simulink model "SpeedGoatLoop_v2"  (R2020b)
settings: Solver=FixedStepAuto  StartTime=0.0  StopTime=60*60*3  RelTol=1e-3
libraries: fl_lib x45, nesl_utility x19, SimscapeFluids_lib x4, speedgoatlib_IO132 x2, slpidlib x1
settings Model: SimulationMode=external  EnablePacing=on  PacingRate=45  ExtModeEnableFloating=off  Creator=cheap  LastModifiedBy=cheap
settings SolverCC: ConcurrentTasks=on  PositivePriorityOrder=on
settings OptimizationCC: BlockReduction=off  OptimizeBlockIOStorage=off
settings DebuggingCC: TasksWithSamePriorityMsg=none
settings HardwareCC: ProdBitPerLong=64  ProdLongLongMode=on  ProdHWDeviceType=Intel->x86-64 (Linux 64)
settings RTWCC: Description=Simulink Real-Time  SystemTargetFile=slrealtime.tlc  TemplateMakefile=slrealtime_default_tmf  Toolchain=Simulink Real-Time Toolchain  BuildConfiguration=Faster Runs  CodeExecutionProfiling=on  TargetLang=C++

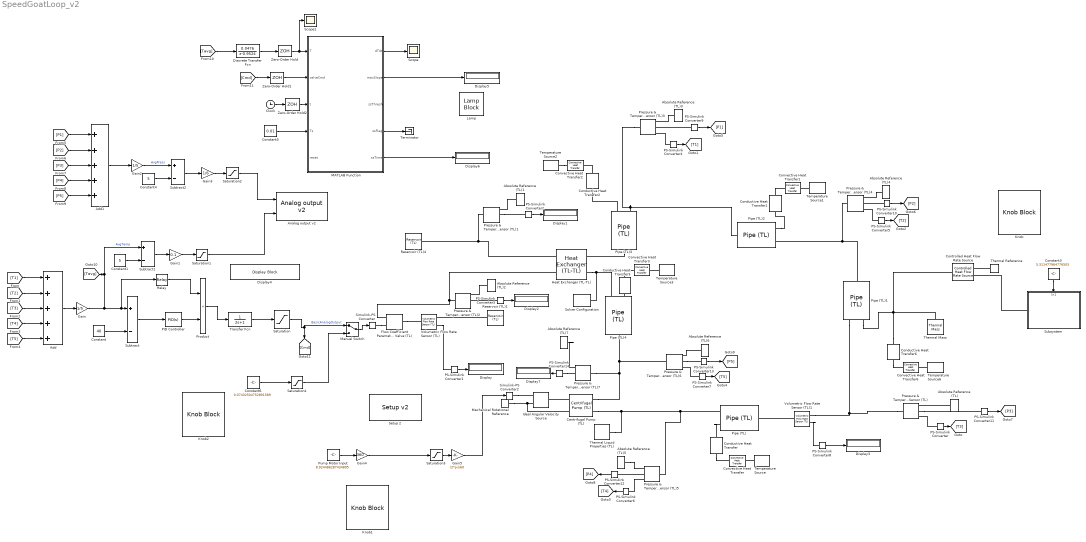
== system SpeedGoatLoop_v2 ==
  Absolute Reference (TL){,1..7} (8 alike) : fl_lib/Thermal Liquid/Elements/Absolute Reference (TL)
      settings: SourceProductBaseCode=SS
  Add : Sum  Inputs=+++++
  Add1 : Sum  Inputs=+++++
  "Analog output v2 " : speedgoatlib_IO132/Analog output v2   parModuleId=1  parSampleTime=-1  parPciSlot=-1  parDacChannels=[1 2]  parDacVoltageRange=[2 2 1 1]  parDacInitValues=[1 1]  parDacReset=[1 1]  parDacSyncOut=1  parDacDmaEnable=0  parDacActiveDmaDevices=1  parDacDmaLatency=2  parDacFrameSize=100
      settings: SourceProductName=Simulink Real-Time: Speedgoat I/O Blockset
  Centrifugal Pump (TL) : SimscapeFluids_lib/Thermal Liquid/Pumps & Motors/Centrifugal Pump (TL)  pump_parameterization=1  mech_orientation=1  flow_rate_1D_TLU=[0 8.33e-5 1.67e-4 2.50e-4 3.33e-4 4.17e-4 5.00e-4 5.83e-4 6.67e-4] m^3/s  head_1D_TLU=[20 19.7 19.0 18.0 16.8 15.2 13.0 10.2 7.5] m  power_1D_TLU=[0 40 80 140 210 290 380 470 550] W  rho_ref_1D=998 kg/m^3  omega_ref_1D=363 rad/s  flow_rate_2D_TLU=[16.67, 23.33, 30, 40, 53.33, 60] lpm  omega_2D_TLU=[2450, 2800, 3150, 3500] rpm  head_2D_TLU=[25, 32.7, 42.5, 50; 24, 31.7, 41, 49; 22.7, 30.5, 39, 47.5; 20, 28, 36, 45; 15.7, 24, 32, 40; 12.5, 21, 29.5, 37.5] m  power_2D_TLU=[.28, .38, .5, .6; .31, .41, .55, .68; .33, .44, .6, .75; .36, .48, .65, .83; .38, .53, .72, .93; .39, .55, .75, .97] kW  rho_ref_2D=920 kg/m^3  omega_threshold=10 rad/s  area=((pi*2)^2)/4 in^2  mdot_A_specify=off  mdot_A_priority=None  mdot_A=1 kg/s  mdot_A_nominal_specify=off  mdot_A_nominal_unit=kg/s  mdot_A_nominal_value=1
      settings: SourceProductBaseCode=SH  InternalSimscapePortConfiguration="{\"Bottom\":[],\"Left\":[{\"id\":\"A\",\"label\":\"A\",\"type\":\"foundation.thermal_liquid.thermal_liquid\"},{\"id\":\"B\",\"label\":\"B\",\"type\":\"foundation.thermal_liquid.thermal_liquid\"}],\"Right\":[{\"id\":\"R\",\"label\":\"R\",\"type\":\"foundation.mechanical.rotational.rotational\"},{\"id\":\"C\",\"label\":\"C\",\"type\":\"foundation.mechanical.rotational.rotational\"}],\"Top\":[]}"
  Clock : Clock
  Conductive Heat Transfer{,1..3,6} (5 alike) : fl_lib/Thermal/Thermal Elements/Conductive Heat Transfer  area=1e-4 m^2  thickness=0.1 m  th_cond=16.2 W/(K*m)  T_specify=off  T_priority=None  T=0 K  T_nominal_specify=off  T_nominal_unit=K  T_nominal_value=1  Q_specify=off  Q_priority=None  Q=0 W  Q_nominal_specify=off  Q_nominal_unit=W  Q_nominal_value=1
  Constant : Constant  Value=40
  Constant1 : Constant  Value=5
  Constant3 : Constant  Value=5.311477964776503
  Constant4 : Constant  Value=5
  Constant5 : Constant  Value=0.01
  Constant6 : Constant  Value=0.07432504752891589
  Controlled Heat Flow Rate Source : fl_lib/Thermal/Thermal Sources/Controlled Heat Flow Rate Source
  Convective Heat Transfer{,1..3} (4 alike) : fl_lib/Thermal/Thermal Elements/Convective Heat Transfer  area=pi*50*(656.10+50.8+179.35+254) mm^2  heat_tr_coeff=10 W/(K*m^2)  T_specify=off  T_priority=None  T=0 K  T_nominal_specify=off  T_nominal_unit=K  T_nominal_value=1  Q_specify=off  Q_priority=None  Q=0 W  Q_nominal_specify=off  Q_nominal_unit=W  Q_nominal_value=1
  Convective Heat Transfer6 : fl_lib/Thermal/Thermal Elements/Convective Heat Transfer  area=pi*50*(6000) mm^2  heat_tr_coeff=10 W/(K*m^2)  T_specify=off  T_priority=None  T=0 K  T_nominal_specify=off  T_nominal_unit=K  T_nominal_value=1  Q_specify=off  Q_priority=None  Q=0 W  Q_nominal_specify=off  Q_nominal_unit=W  Q_nominal_value=1
  Discrete Transfer Fcn : DiscreteTransferFcn  Numerator=[0.0476]  Denominator=[1 -0.9524]  SampleTime=0.01
  Display{,1..3,5..7} (7 alike) : Display
  Display4 : DisplayBlock  LabelPosition=Hide  Format=short  Transparency=1
  Flow Coefficient Parameterized Valve (TL) : SimscapeFluids_lib/Thermal Liquid/Valves & Orifices/Flow Coefficient Parameterized Valve (TL)  flow_coeff_spec=fluids.thermal_liquid.valves.enum.flow_coeff_spec.cv  Cv_max=1  Cv_min=1e-4  Kv_max=1  Kv_min=1e-4  valve_character=fluids.thermal_liquid.valves.enum.valve_opening_spec.linear  rangeability=50  alpha=2  area=((0.75*pi)^2)/4 in^2  length=3 in  Re_c=12  smoothing_factor=0.02  opening_dynamic=simscape.enum.onoff.off  tau=0.1 s  mdot_A_specify=off  mdot_A_priority=None  mdot_A=1 kg/s  mdot_A_nominal_specify=off  mdot_A_nominal_unit=kg/s  mdot_A_nominal_value=1  area_dynamic_specify=off  area_dynamic_priority=High  area_dynamic=1e-10 m^2  area_dynamic_nominal_specify=off  area_dynamic_nominal_unit=m^2  area_dynamic_nominal_value=1
      settings: SourceProductBaseCode=SH  InternalSimscapePortConfiguration="{\"Bottom\":[],\"Left\":[{\"id\":\"A\",\"label\":\"A\",\"type\":\"foundation.thermal_liquid.thermal_liquid\"},{\"id\":\"L\",\"label\":\"L\",\"type\":\"input\"}],\"Right\":[{\"id\":\"B\",\"label\":\"B\",\"type\":\"foundation.thermal_liquid.thermal_liquid\"}],\"Top\":[]}"
  Gain : Gain  Gain=1/5
  Gain1 : Gain  Gain=0.1
  Gain2 : Gain  Gain=1/5
  Gain3 : Gain  Gain=1/6
  Gain4 : Gain  Gain=360
  Gain5 : Gain  Gain=(2*pi)/60
  Heat Exchanger (TL-TL) : SimscapeFluids_lib/Fluid Network Interfaces/Heat Exchangers/Heat Exchanger (TL-TL)  hex_type=fluids.interfaces.enum.flow_arrangement_spec.shell_tube  cross_type=fluids.interfaces.enum.cross_flow_heat_exchanger_TL_TL_spec.mixed_mixed  shell_num=1  NTU_TLU=[.5, 1, 2, 3, 4, 5]  CR_TLU=[0, .25, .5, .75, 1]  eff_TLU=[.3, .3, .3, .3, .3; .6, .55, .5, .47, .43; .85, .76, .68, .61, .55; .94, .83, .72, .65, .58; .98, .86, .75, .66, .58; .99, .86, .75, .66, .58]  wall_thermal_dynamics=simscape.enum.onoff.on  thermal_mass_wall=447 J/K  R_wall=1.984E-3 K/W  min_flow_area_1=1.16E-3 m^2  Dh_press_1=0.00451 m  liquid_volume_1=3E-3 m^3  Re_lam_1=2000  Re_tur_1=4000  pressure_loss_spec_1=fluids.interfaces.enum.pressure_loss_spec.constant  min_flow_area_2=9.19E-4 m^2  Dh_press_2=0.004572 m  liquid_volume_2=8.41E-4 m^3  Re_lam_2=2000  Re_tur_2=4000  pressure_loss_spec_2=fluids.interfaces.enum.pressure_loss_spec.tube_correlation  pressure_loss_coeff_1=0.1  length_press_1=1 m  length_add_1=0.1 m  roughness_1=15e-6 m  Re_friction_TLU_1=[400, 1000, 1500, 3000, 4000, 6000, 10000, 20000, 40000, 60000, 100000, 100000000]  friction_factor_TLU_1=[.264, .112, .071, .0417, .0387, .0268, .025, .0232, .0226, .022, .0214, .0214]  shape_factor_1=64  Re_Euler_TLU_1=[50, 500, 1000, 2000]  Euler_TLU_1=[4.4505, .6864, .4791, .3755]  pressure_loss_coeff_2=0.1  length_press_2=0.9144 m  length_add_2=0.4 m  roughness_2=15e-6 m  Re_friction_TLU_2=[400, 1000, 1500, 3000, 4000, 6000, 10000, 20000, 40000, 60000, 100000, 100000000]  friction_factor_TLU_2=[.264, .112, .071, .0417, .0387, .0268, .025, .0232, .0226, .022, .0214, .0214]  shape_factor_2=64  Re_Euler_TLU_2=[50, 500, 1000, 2000]  Euler_TLU_2=[4.4505, .6864, .4791, .3755]  heat_transfer_spec_1=fluids.interfaces.enum.heat_transfer_spec.constant  heat_transfer_spec_2=fluids.interfaces.enum.heat_transfer_spec.tube_correlation  heat_coeff_1=100 W/(m^2 * K)  length_heat_1=1 m  Nu_lam_1=3.66  Re_Colburn_TLU_1=[100, 150, 1000]  Colburn_factor_TLU_1=[.019, .013, .002]  Re_Nu_TLU_1=[100, 150, 1000]  Pr_Nu_TLU_1=[1, 10]  Nu_TLU_1=[3.72, 4.21; 3.75, 4.44; 4.21, 7.15]  heat_coeff_2=100 W/(m^2 * K)  length_heat_2=0.9144 m  Nu_lam_2=3.66  Re_Colburn_TLU_2=[100, 150, 1000]  Colburn_factor_TLU_2=[.019, .013, .002]  Re_Nu_TLU_2=[100, 150, 1000]  Pr_Nu_TLU_2=[1, 10]  Nu_TLU_2=[3.72, 4.21; 3.75, 4.44; 4.21, 7.15]  heat_transfer_area_1=1.022 m^2  fouling_factor_1=1e-4 m^2*K/W  min_heat_coeff_1=3000 W/(m^2 * K)  heat_transfer_area_2=0.735 m^2  fouling_factor_2=1e-4 m^2*K/W  min_heat_coeff_2=10000 W/(m^2 * K)  dynamic_compressibility_1=simscape.enum.onoff.on  T0_1=10 degC  p0_1=60 psi  dynamic_compressibility_2=simscape.enum.onoff.on  T0_2=24 degC  p0_2=30 psi  mdot1_TLU=[.3, .5, .6, .7, 1, 1.4, 1.9, 2.3] kg/s  mdot2_TLU=[.3, .5, 1, 1.3, 1.7, 2, 2.6, 3.3] kg/s  SD_TLU=[.324, .3533, .404, .4253, .4333, .4373, .4453, .4533; .3813, .424, .496, .5307, .544, .5547, .5693, .5787; .4267, .4827, .5813, .6173, .6413, .6573, .672, .6827; .4613, .528, .64, .6987, .7267, .7467, .7707, .7853; .5533, .6467, .8227, .928, .9853, 1.0187, 1.0653, 1.0973; .58, .688, .8853, 1.0147, 1.08, 1.124, 1.176, 1.2147; .624, .7467, .992, 1.148, 1.244, 1.304, 1.3773, 1.4267; .656, .7907, 1.0667, 1.26, 1.376, 1.452, 1.548, 1.612] kW/K  Q_check=fluids.interfaces.enum.SD_max_check.warning  mdot_dp_TLU_1=[.3, .5, 1, 1.5, 2, 2.5] kg/s  p_diff_TLU_1=[3, 5, 10, 25, 35, 50] * 1e-3 MPa  T_ref_in_1=293.15 K  p_ref_in_1=0.101325 MPa  mdot_threshold_1=1e-3 kg/s  area_1=0.01 m^2  mdot_dp_TLU_2=[.3, .5, 1, 1.5, 2, 2.5] kg/s  p_diff_TLU_2=[3, 5, 10, 25, 35, 50] * 1e-3 MPa  T_ref_in_2=293.15 K  p_ref_in_2=0.101325 MPa  mdot_threshold_2=1e-3 kg/s  area_2=0.01 m^2
      settings: SourceProductBaseCode=SH  InternalSimscapePortConfiguration="{\"Bottom\":[],\"Left\":[{\"id\":\"A1\",\"label\":\"A1\",\"type\":\"foundation.thermal_liquid.thermal_liquid\"},{\"id\":\"B1\",\"label\":\"B1\",\"type\":\"foundation.thermal_liquid.thermal_liquid\"}],\"Right\":[{\"id\":\"A2\",\"label\":\"A2\",\"type\":\"foundation.thermal_liquid.thermal_liquid\"},{\"id\":\"B2\",\"label\":\"B2\",\"type\":\"foundation.thermal_liquid.thermal_liquid\"}],\"Top\":[]}"
  Ideal Angular Velocity Source : fl_lib/Mechanical/Mechanical Sources/Ideal Angular Velocity Source
  Knob : KnobBlock  ScaleMax=20
  Knob1 : KnobBlock  ScaleMax=10
  Knob2 : KnobBlock  ScaleMax=1
  Lamp : LampBlock
  MATLAB Function : MATLAB Function  TreatAsAtomicUnit=on
  Manual Switch : ManualSwitch
  Mechanical Rotational Reference : fl_lib/Mechanical/Rotational Elements/Mechanical Rotational Reference
  PID Controller : slpidlib/PID Controller  Controller=PID  Form=Parallel  TimeDomain=Continuous-time  UseExternalTs=off  SampleTime=-1  IntegratorMethod=Forward Euler  FilterMethod=Forward Euler  ControllerParametersSource=internal  P=0.015  I=2e-5  D=0  UseFilter=on  N=100  TunerSelectOption=Transfer Function Based (PID Tuner App)  InitialConditionSource=internal  InitialConditionForIntegrator=0  InitialConditionForFilter=0  DifferentiatorICPrevScaledInput=0  ExternalReset=none  TrackingMode=off  Kt=1  LimitOutput=on  SatLimitsSource=internal  UpperSaturationLimit=1  LowerSaturationLimit=0  LinearizeAsGain=on  AntiWindupMode=clamping  Kb=1  POutMin=[]  POutMax=[]  IOutMin=[]  IOutMax=[]  DOutMin=[]  DOutMax=[]  NOutMin=[]  NOutMax=[]  SumOutMin=[]  SumOutMax=[]  SaturationOutMin=[]  SaturationOutMax=[]  PParamMin=[]  PParamMax=[]  IParamMin=[]  IParamMax=[]  DParamMin=[]  DParamMax=[]  NParamMin=[]  NParamMax=[]  KbParamMin=[]  KbParamMax=[]  KtParamMin=[]  KtParamMax=[]  KbOutMin=[]  KbOutMax=[]  KtOutMin=[]  KtOutMax=[]  IntegratorOutMin=[]  IntegratorOutMax=[]  FilterOutMin=[]  FilterOutMax=[]  SumI1OutMin=[]  SumI1OutMax=[]  SumI2OutMin=[]  SumI2OutMax=[]  SumI3OutMin=[]  SumI3OutMax=[]  SumI4OutMin=[]  SumI4OutMax=[]  SumDOutMin=[]  SumDOutMax=[]  DifferentiatorOutMin=[]  DifferentiatorOutMax=[]  FilterDiffOutCoefMin=[]  FilterDiffOutCoefMax=[]  ReciprocalOutMin=[]  ReciprocalOutMax=[]  SumDenOutMin=[]  SumDenOutMax=[]  SumNumOutMin=[]  SumNumOutMax=[]  DivideOutMin=[]  DivideOutMax=[]  UdiffTsProdOutMin=[]  UdiffTsProdOutMax=[]  NTsProdOutMin=[]  NTsProdOutMax=[]  UintegralTsProdOutMin=[]  UintegralTsProdOutMax=[]  UngainTsProdOutMin=[]  UngainTsProdOutMax=[]  IntegratorContinuousStateAttributes=''  IntegratorStateMustResolveToSignalObject=off  IntegratorRTWStateStorageClass=Auto  FilterContinuousStateAttributes=''  FilterStateMustResolveToSignalObject=off  FilterRTWStateStorageClass=Auto  ParallelPVariant=InternalParameters  IdealPVariant=Disabled  IVariant=InternalParameters  DVariant=InternalParameters  IntegratorVariant=Continuous  SatVariant=Enabled  AWVariant=ContClampingParallel  PCopyVariant=Disabled  TRVariant=Disabled  FdbkBlocksVariant=Forward  IdealPFdbkVariant=Disabled  SatFdbkVariant=Disabled  DerivativeFilterVariant=ContFilter  NVariant=InternalParameters  NCopyVariant=Disabled  FilterICVariant=InternalICsFilter  IntegratorICVariant=InternalICs  ExternalResetVariant=Disabled  TRSumVariant=Passthrough  SumFdbkVariant=Disabled  SumVariant=Sum_PID  TsampFilterVariant=InternalTs  TsampNgainVariant=Passthrough  TsampIntegralVariant=Passthrough  ExternalSaturationOutDataTypeStr=Inherit: Same as second input
  PS-Simulink Converter{,4..7} (5 alike) : nesl_utility/PS-Simulink Converter  PhysicalDomain=network_engine_domain  SubClassName=ps_output  LeftPortType=input  RightPortType=output  PseudoPeriodic=off  Frequencies=[]  Unit=degC  AffineConversion=on
  PS-Simulink Converter1 : nesl_utility/PS-Simulink Converter  PhysicalDomain=network_engine_domain  SubClassName=ps_output  LeftPortType=input  RightPortType=output  PseudoPeriodic=off  Frequencies=[]  Unit=gpm  AffineConversion=on
  PS-Simulink Converter{2,9..14} (7 alike) : nesl_utility/PS-Simulink Converter  PhysicalDomain=network_engine_domain  SubClassName=ps_output  LeftPortType=input  RightPortType=output  PseudoPeriodic=off  Frequencies=[]  Unit=psi  AffineConversion=on
  PS-Simulink Converter3 : nesl_utility/PS-Simulink Converter  PhysicalDomain=network_engine_domain  SubClassName=ps_output  LeftPortType=input  RightPortType=output  PseudoPeriodic=off  Frequencies=[]  Unit=inherit  AffineConversion=off
  PS-Simulink Converter8 : nesl_utility/PS-Simulink Converter  PhysicalDomain=network_engine_domain  SubClassName=ps_output  LeftPortType=input  RightPortType=output  PseudoPeriodic=off  Frequencies=[]  Unit=gpm  AffineConversion=on
  Pipe (TL) : fl_lib/Thermal Liquid/Elements/Pipe (TL)  length=572+698.5+113+656.1+50.8+179.35+254 mm  area=((1.7*pi)^2)/4 in^2  Dh=1.5 in  length_add=1 m  roughness=15e-6 m  Re_lam=2000  Re_tur=4000  shape_factor=64  Nu_lam=3.66  dynamic_compressibility=simscape.enum.onoff.on  inertia=simscape.enum.onoff.off  p0=30 psi  T0=24 degC  mdot0=0 kg/s
      settings: SourceProductBaseCode=SS
  Pipe (TL)1 : fl_lib/Thermal Liquid/Elements/Pipe (TL)  length=1666.08+113 mm  area=((50*pi)^2)/4 mm^2  Dh=1.5 in  length_add=1 m  roughness=15e-6 m  Re_lam=2000  Re_tur=4000  shape_factor=64  Nu_lam=3.66  dynamic_compressibility=simscape.enum.onoff.on  inertia=simscape.enum.onoff.off  p0=30 psi  T0=24 degC  mdot0=0 kg/s
      settings: SourceProductBaseCode=SS
  Pipe (TL)2 : fl_lib/Thermal Liquid/Elements/Pipe (TL)  length=322.66+283.65+665.16+113+331.45+863.6 mm  area=((1.7*pi)^2)/4 in^2  Dh=1.5 in  length_add=1 m  roughness=15e-6 m  Re_lam=2000  Re_tur=4000  shape_factor=64  Nu_lam=3.66  dynamic_compressibility=simscape.enum.onoff.on  inertia=simscape.enum.onoff.off  p0=30 psi  T0=24 degC  mdot0=0 kg/s
      settings: SourceProductBaseCode=SS
  Pipe (TL)3 : fl_lib/Thermal Liquid/Elements/Pipe (TL)  length=211.02+1024.8+164.52+317.72 mm  area=((1.7*pi)^2)/4 in^2  Dh=1.5 in  length_add=1 m  roughness=15e-6 m  Re_lam=2000  Re_tur=4000  shape_factor=64  Nu_lam=3.66  dynamic_compressibility=simscape.enum.onoff.on  inertia=simscape.enum.onoff.off  p0=30 psi  T0=24 degC  mdot0=0 kg/s
      settings: SourceProductBaseCode=SS
  Pipe (TL)4 : fl_lib/Thermal Liquid/Elements/Pipe (TL)  length=211.02+1024.8+164.52+317.72 mm  area=((1.7*pi)^2)/4 in^2  Dh=1.5 in  length_add=1 m  roughness=15e-6 m  Re_lam=2000  Re_tur=4000  shape_factor=64  Nu_lam=3.66  dynamic_compressibility=simscape.enum.onoff.on  inertia=simscape.enum.onoff.off  p0=30 psi  T0=24 degC  mdot0=0 kg/s
      settings: SourceProductBaseCode=SS
  Pressure & Temperature Sensor (TL){,1..7} (8 alike) : fl_lib/Thermal Liquid/Sensors/Pressure & Temperature Sensor (TL)
      settings: SourceProductBaseCode=SS  InternalSimscapePortConfiguration="{\"Bottom\":[],\"Left\":[{\"id\":\"A\",\"label\":\"A\",\"type\":\"foundation.thermal_liquid.thermal_liquid\"}],\"Right\":[{\"id\":\"B\",\"label\":\"B\",\"type\":\"foundation.thermal_liquid.thermal_liquid\"},{\"id\":\"P\",\"label\":\"P\",\"type\":\"output\"},{\"id\":\"T\",\"label\":\"T\",\"type\":\"output\"}],\"Top\":[]}"
  Product : Product
  Pump Motor Input : Constant  Value=8.924486287434895
  Relay : Relay  OnSwitchValue=38  OffSwitchValue=36
  Reservoir (TL)1 : fl_lib/Thermal Liquid/Elements/Reservoir (TL)  pressure_spec=foundation.enum.pressure_spec.atmospheric  reservoir_pressure=0.101325 MPa  reservoir_temperature=10 degC  area=((pi*1.5)^2)/4 in^2
      settings: SourceProductBaseCode=SS
  Reservoir (TL)4 : fl_lib/Thermal Liquid/Elements/Reservoir (TL)  pressure_spec=foundation.enum.pressure_spec.specified  reservoir_pressure=60 psi  reservoir_temperature=10 degC  area=((pi*1.5)^2)/4 in^2
      settings: SourceProductBaseCode=SS
  Saturation : Saturate  UpperLimit=0.98  LowerLimit=0.0002
  Saturation1 : Saturate  UpperLimit=10  LowerLimit=0
  Saturation2 : Saturate  UpperLimit=90  LowerLimit=20
  Saturation3 : Saturate  UpperLimit=3600  LowerLimit=0
  Saturation4 : Saturate  UpperLimit=0.98  LowerLimit=0.02
  Scope : Scope
  Scope1 : Scope
  "Setup 2 " : speedgoatlib_IO132/Setup v2   parPciSlot=-1  parModuleId=1  parInterModuleSync=None  parConvClockBaseRate=20MHz  parConvClock1Divider=20000  parConvClock2Divider=20000  parFrameTriggerEnable=off  parFrameTriggerDivider=10  parConvClock1BaseRate=1  parConvClock2BaseRate=1  parFrameTriggerClock=1  parAdcChannels=[1]  parAdcRange1=+-10V  parAdcOversampling1=None  parAdcAutoCorrection=on  parAdcContSampling=off  parAdcVoltageRange=2  parAdcOversamplRate=1  parAdcDmaEnable=off  parAdcDmaClock=Clock 1  parAdcFrameSize_=100  parAdcSampleTime_=-1  parAdcActiveDmaDevices=[1]  parAdcFrameTriggerEnable=0  parAdcFrameSize=100  parAdcSampleTime=0.1  parDacChannels=[1 2]  parDacInitValues=1  parDacReset=1  parDacRange1=0-10V  parDacRange2=0-10V  parDacRange3=0-5V  parDacRange4=0-5V  parDacVoltageRange=[2 2 1 1]  parDacAutoCorrection=on  parDacSyncOut=on  parDacDmaEnable=off  parDacDmaLatency=Until next frame  parDacDmaClock=Clock 1  parDacFrameSize_=100  parDacSampleTime_=-1  parDacActiveDmaDevices=[1]  parDacFrameTriggerEnable=0  parDacFrameSize=100  parDacSampleTime=0.1  parDoChannels=[1 2]  parDoInitValues=0  parDoReset=1  parDiChannels=[3 4]  parDiDebounceEnable=off  parDiDebounceTime=0  parDiDebounceValue=0  parDioPullRefFront=Pull-up 3.3V  parDioPullRefRear=Floating
      settings: SourceProductName=Simulink Real-Time: Speedgoat Library
  Simulink-PS Converter : nesl_utility/Simulink-PS Converter  PhysicalDomain=network_engine_domain  SubClassName=ps_input  LeftPortType=input  RightPortType=output  PseudoPeriodic=off  Frequencies=[]  NoiseDistribution=none  NoiseParameters=[]  Unit=1  AffineConversion=off  FilteringAndDerivatives=provide  SimscapeFilterOrder=1  InputFilterTimeConstant=0.001  UdotUserProvided=0
  Simulink-PS Converter2 : nesl_utility/Simulink-PS Converter  PhysicalDomain=network_engine_domain  SubClassName=ps_input  LeftPortType=input  RightPortType=output  PseudoPeriodic=off  Frequencies=[]  NoiseDistribution=none  NoiseParameters=[]  Unit=1  AffineConversion=off  FilteringAndDerivatives=provide  SimscapeFilterOrder=1  InputFilterTimeConstant=0.001  UdotUserProvided=0
  Solver Configuration : nesl_utility/Solver Configuration  PhysicalDomain=network_engine_domain  SubClassName=solver  LeftPortType=input  RightPortType=generic  Tones=[]  Harmonics=[]  SimulateNoise=off  Profile=off  UseLocalSampling=off  EnableSwitchedLinearOptims=on  FrequencyDomain=off  UseCCode=off  RelTol=0.001  AbsTol=1e-06  MinStep=1e-09  ToWorkspace=off  RevertToSquareIcSolve=off  NumHomotopyIterations=100  PhasorMode=off  PhasorModeNumHarmonics=1  DoDC=on  ResidualTolerance=1e-09  UseLocalSolver=on  LocalSolverChoice=NE_BACKWARD_EULER_ADVANCER  LocalSolverSampleTime=0.01  DoFixedCost=on  MaxNonlinIter=3  MaxModeIter=2  ComputeImpulses=off  ImpulseIterations=2  LinearAlgebra=auto  EquationFormulation=NE_TIME_EF  DelaysMemoryBudget=1024  AutomaticFiltering=on  FilteringTimeConstant=0.001  PartitionStorageMethod=AS_NEEDED  PartitionMemoryBudget=1024  PartitionMethod=ROBUST
  Subsystem : Subsystem
      settings: PortSchema="{\"entries\":[{\"content\":{\"sides\":[{\"content\":{\"connectorIds\":[\"LConn1\"]},\"type\":\"ConnectorPlacement.EquallySpacedRectSide\",\"uuid\":\"fb919825-1b2f-4c31-9805-0967e26cfa90\"},{\"content\":{\"side\":\"RIGHT\"},\"type\":\"ConnectorPlacement.EquallySpacedRectSide\",\"uuid\":\"9136b45b-edcb-43b5-a0c1-cf6d919585f5\"},{\"content\":{\"connectorIds\":[\"In1\"],\"side\":\"TOP\"},\"type\":\"ConnectorPlacement.EquallySpacedRectSide\",\"uuid\":\"eaf0a6cf-ad87-41c1-a56b-7e33ba526407\"}]},\"type\":\"ConnectorPlacement.EquallySpacedConnector\",\"uuid\":\"77377397-7f65-431b-b464-9c22985d1642\"}],\"packageUris\":[\"http://schema.mathworks.com/mf0/Connector/R2020b\"],\"version\":\"1.0\"}"
  Subtract : Sum  Inputs=+-
  Subtract1 : Sum  Inputs=+-
  Subtract2 : Sum  Inputs=+-
  Temperature Source{,1..3,6} (5 alike) : fl_lib/Thermal/Thermal Sources/Temperature Source  temperature=293.15 K
  Terminator : Terminator
  Thermal Liquid Properties (TL) : SimscapeFluids_lib/Thermal Liquid/Utilities/Thermal Liquid Properties (TL)  fluid_list=fluids.thermal_liquid.utilities.enum.thermal_liquid_fluid_list.water  concentration_param_EG=fluids.thermal_liquid.utilities.enum.thermal_liquid_concentration.volume_fraction  concentration_param_PG=fluids.thermal_liquid.utilities.enum.thermal_liquid_concentration.volume_fraction  c_mass_SW=3.5e-3  c_mass_EG=0.1  c_mass_PG=0.1  c_mass_GL=0.1  c_vol_EG=0.1  c_vol_PG=0.1  beta_const_EG=2.1791 GPa  beta_const_PG=2.1791 GPa  beta_const_GL=2.1791 GPa  p_min_EG=0.01 MPa  p_min_PG=0.01 MPa  p_min_GL=0.01 MPa  p_max_EG=50 MPa  p_max_PG=50 MPa  p_max_GL=50 MPa  p_atm=0.101325 MPa
      settings: SourceProductBaseCode=SH
  Thermal Mass : fl_lib/Thermal/Thermal Elements/Thermal Mass  mass=3 kg  sp_heat=450 J/(K*kg)  T_specify=off  T_priority=High  T=300 K  T_nominal_specify=off  T_nominal_unit=K  T_nominal_value=1  Q_specify=off  Q_priority=None  Q=0 W  Q_nominal_specify=off  Q_nominal_unit=W  Q_nominal_value=1
  Thermal Reference : fl_lib/Thermal/Thermal Elements/Thermal Reference
  Transfer Fcn : TransferFcn  Denominator=[2 1]
  Volumetric Flow Rate Sensor (TL) : fl_lib/Thermal Liquid/Sensors/Volumetric Flow Rate Sensor (TL)
      settings: SourceProductBaseCode=SS  InternalSimscapePortConfiguration="{\"Bottom\":[],\"Left\":[{\"id\":\"A\",\"label\":\"A\",\"type\":\"foundation.thermal_liquid.thermal_liquid\"}],\"Right\":[{\"id\":\"B\",\"label\":\"B\",\"type\":\"foundation.thermal_liquid.thermal_liquid\"},{\"id\":\"V\",\"label\":\"V\",\"type\":\"output\"}],\"Top\":[]}"
  Volumetric Flow Rate Sensor (TL)1 : fl_lib/Thermal Liquid/Sensors/Volumetric Flow Rate Sensor (TL)
      settings: SourceProductBaseCode=SS  InternalSimscapePortConfiguration="{\"Bottom\":[],\"Left\":[{\"id\":\"A\",\"label\":\"A\",\"type\":\"foundation.thermal_liquid.thermal_liquid\"}],\"Right\":[{\"id\":\"B\",\"label\":\"B\",\"type\":\"foundation.thermal_liquid.thermal_liquid\"},{\"id\":\"V\",\"label\":\"V\",\"type\":\"output\"}],\"Top\":[]}"
  Zero-Order Hold : ZeroOrderHold  SampleTime=0.01
  Zero-Order Hold1 : ZeroOrderHold  SampleTime=0.01
  Zero-Order Hold2 : ZeroOrderHold  SampleTime=0.01
  wires:
  PS-Simulink Converter12/1 -> [P4]
  Saturation2/1 -> "Analog output v2 "/1
  Constant/1 -> Subtract/2
  [T5] -> Add/5
  PS-Simulink Converter7/1 -> [T5]
  [T4] -> Add/4
  [T2] -> Add/2
  PS-Simulink Converter6/1 -> [T4]
  PS-Simulink Converter5/1 -> [T2]
  Zero-Order Hold2/1 -> MATLAB Function/3(t)
  Subtract/1 -> PID Controller/1
  Gain/1 -> [Tavg], Subtract1/1, Relay/1, Subtract/1  "AvgTemp"
  PS-Simulink Converter/1 -> [T3]
  Saturation/1 -> Manual Switch/1, [Cmd]  "BasicAnalogOutput"
  PS-Simulink Converter1/1 -> Display/1
  PS-Simulink Converter2/1 -> Display1/1
  PS-Simulink Converter3/1 -> Display2/1
  Transfer Fcn/1 -> Saturation/1
  Subtract1/1 -> Gain1/1
  Constant1/1 -> Subtract1/2
  Relay/1 -> Product/1
  PID Controller/1 -> Product/2
  PS-Simulink Converter4/1 -> [T1]
  PS-Simulink Converter8/1 -> Display3/1
  [P1] -> Add1/1
  Gain3/1 -> Saturation2/1
  MATLAB Function/2(maxSlope) -> Display5/1
  Zero-Order Hold/1 -> Scope1/1, MATLAB Function/1(T)
  Discrete Transfer Fcn/1 -> Zero-Order Hold/1
  MATLAB Function/4(ssFlag) -> Terminator/1
  [Tavg] -> Discrete Transfer Fcn/1
  Constant3/1 -> Subsystem/1(In1)
  Add/1 -> Gain/1
  [T1] -> Add/1
  [Cmd] -> Zero-Order Hold1/1
  [T3] -> Add/3
  Constant5/1 -> MATLAB Function/4(Ts)
  Saturation1/1 -> "Analog output v2 "/2
  MATLAB Function/5(ssTime) -> Display6/1
  Subtract2/1 -> Gain3/1
  Product/1 -> Transfer Fcn/1
  Add1/1 -> Gain2/1
  Gain1/1 -> Saturation1/1
  [P2] -> Add1/2
  [P4] -> Add1/4
  MATLAB Function/1(dTdt) -> Scope/1
  Clock/1 -> Zero-Order Hold2/1
  Zero-Order Hold1/1 -> MATLAB Function/2(valveCmd)
  Gain2/1 -> Subtract2/1  "AvgPress"
  Constant4/1 -> Subtract2/2
  PS-Simulink Converter9/1 -> [P1]
  [P5] -> Add1/5
  PS-Simulink Converter13/1 -> [P5]
  PS-Simulink Converter10/1 -> [P2]
  PS-Simulink Converter11/1 -> [P3]
  [P3] -> Add1/3
  Pump Motor Input/1 -> Gain4/1
  Gain4/1 -> Saturation3/1
  Saturation3/1 -> Gain5/1
  Gain5/1 -> Simulink-PS Converter2/1
  Manual Switch/1 -> Simulink-PS Converter/1
  Constant6/1 -> Saturation4/1
  Saturation4/1 -> Manual Switch/2
  PS-Simulink Converter14/1 -> Display7/1
  connections:
  Pipe (TL)2/LConn1 -- Pipe (TL)1/RConn1 -- Pressure & Temperature Sensor (TL)4/LConn1
  Conductive Heat Transfer6/LConn1 -- Pipe (TL)1/LConn2 -- Thermal Mass/LConn1 -- Controlled Heat Flow Rate Source/LConn1
  Pressure & Temperature Sensor (TL)5/LConn1 -- Thermal Liquid Properties (TL)/RConn1 -- Centrifugal Pump (TL)/LConn2 -- Pipe (TL)/LConn1
  Pressure & Temperature Sensor (TL)3/LConn1 -- Pipe (TL)2/RConn1 -- Pipe (TL)3/LConn1
  Pressure & Temperature Sensor (TL)/LConn1 -- Pipe (TL)1/LConn1 -- Volumetric Flow Rate Sensor (TL)1/RConn1
  Pressure & Temperature Sensor (TL)1/LConn1 -- Reservoir (TL)4/LConn1 -- Heat Exchanger (TL-TL)/LConn1
  Pressure & Temperature Sensor (TL)2/LConn1 -- Heat Exchanger (TL-TL)/LConn2 -- Flow Coefficient Parameterized Valve (TL)/LConn1
  Pipe (TL)3/LConn2 -- Conductive Heat Transfer2/LConn1
  Absolute Reference (TL)/LConn1 -- Pressure & Temperature Sensor (TL)/RConn1
  Volumetric Flow Rate Sensor (TL)1/RConn2 -- PS-Simulink Converter8/LConn1
  Pressure & Temperature Sensor (TL)/RConn2 -- PS-Simulink Converter11/LConn1
  PS-Simulink Converter4/LConn1 -- Pressure & Temperature Sensor (TL)3/RConn3
  Subsystem/LConn1 -- Controlled Heat Flow Rate Source/RConn1
  Conductive Heat Transfer6/RConn1 -- Convective Heat Transfer6/LConn1
  Pressure & Temperature Sensor (TL)1/RConn2 -- PS-Simulink Converter2/LConn1
  PS-Simulink Converter7/LConn1 -- Pressure & Temperature Sensor (TL)6/RConn3
  Absolute Reference (TL)1/LConn1 -- Pressure & Temperature Sensor (TL)1/RConn1
  Pipe (TL)/LConn2 -- Conductive Heat Transfer/LConn1
  Absolute Reference (TL)6/LConn1 -- Pressure & Temperature Sensor (TL)6/RConn1
  Absolute Reference (TL)3/LConn1 -- Pressure & Temperature Sensor (TL)3/RConn1
  Temperature Source2/LConn1 -- Convective Heat Transfer2/RConn1
  Absolute Reference (TL)5/LConn1 -- Pressure & Temperature Sensor (TL)5/RConn1
  Temperature Source/LConn1 -- Convective Heat Transfer/RConn1
  Conductive Heat Transfer/RConn1 -- Convective Heat Transfer/LConn1
  Temperature Source6/LConn1 -- Convective Heat Transfer6/RConn1
  Volumetric Flow Rate Sensor (TL)1/LConn1 -- Pipe (TL)/RConn1
  Temperature Source1/LConn1 -- Convective Heat Transfer1/RConn1
  Pressure & Temperature Sensor (TL)5/RConn2 -- PS-Simulink Converter12/LConn1
  Conductive Heat Transfer2/RConn1 -- Convective Heat Transfer2/LConn1
  PS-Simulink Converter/LConn1 -- Pressure & Temperature Sensor (TL)/RConn3
  PS-Simulink Converter5/LConn1 -- Pressure & Temperature Sensor (TL)4/RConn3
  Absolute Reference (TL)4/LConn1 -- Pressure & Temperature Sensor (TL)4/RConn1
  Pressure & Temperature Sensor (TL)2/RConn2 -- PS-Simulink Converter3/LConn1
  Thermal Reference/LConn1 -- Controlled Heat Flow Rate Source/RConn2
  Flow Coefficient Parameterized Valve (TL)/RConn1 -- Volumetric Flow Rate Sensor (TL)/LConn1
  Pipe (TL)2/LConn2 -- Conductive Heat Transfer1/LConn1
  PS-Simulink Converter9/LConn1 -- Pressure & Temperature Sensor (TL)3/RConn2
  PS-Simulink Converter6/LConn1 -- Pressure & Temperature Sensor (TL)5/RConn3
  Volumetric Flow Rate Sensor (TL)/RConn2 -- PS-Simulink Converter1/LConn1
  Pipe (TL)3/RConn1 -- Heat Exchanger (TL-TL)/RConn1
  PS-Simulink Converter10/LConn1 -- Pressure & Temperature Sensor (TL)4/RConn2
  Conductive Heat Transfer1/RConn1 -- Convective Heat Transfer1/LConn1
  Reservoir (TL)1/LConn1 -- Volumetric Flow Rate Sensor (TL)/RConn1
  Pressure & Temperature Sensor (TL)6/RConn2 -- PS-Simulink Converter13/LConn1
  Absolute Reference (TL)2/LConn1 -- Pressure & Temperature Sensor (TL)2/RConn1
  Mechanical Rotational Reference/LConn1 -- Centrifugal Pump (TL)/RConn2 -- Ideal Angular Velocity Source/RConn2
  Centrifugal Pump (TL)/RConn1 -- Ideal Angular Velocity Source/LConn1
  Simulink-PS Converter2/RConn1 -- Ideal Angular Velocity Source/RConn1
  Simulink-PS Converter/RConn1 -- Flow Coefficient Parameterized Valve (TL)/LConn2
  Heat Exchanger (TL-TL)/RConn2 -- Solver Configuration/RConn1 -- Pipe (TL)4/LConn1
  Temperature Source3/LConn1 -- Convective Heat Transfer3/RConn1
  Conductive Heat Transfer3/RConn1 -- Convective Heat Transfer3/LConn1
  Conductive Heat Transfer3/LConn1 -- Pipe (TL)4/LConn2
  Absolute Reference (TL)7/LConn1 -- Pressure & Temperature Sensor (TL)7/RConn1
  PS-Simulink Converter14/LConn1 -- Pressure & Temperature Sensor (TL)7/RConn2
  Centrifugal Pump (TL)/LConn1 -- Pipe (TL)4/RConn1 -- Pressure & Temperature Sensor (TL)6/LConn1 -- Pressure & Temperature Sensor (TL)7/LConn1

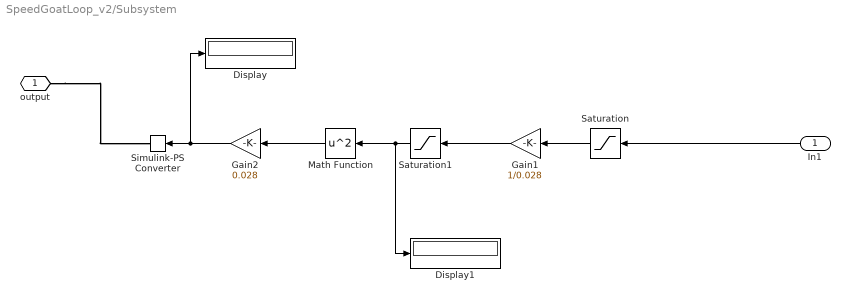
== system SpeedGoatLoop_v2/Subsystem ==
  In1 : Inport
  Display : Display
  Display1 : Display
  Gain1 : Gain  Gain=1/0.028
  Gain2 : Gain  Gain=0.028
  Math Function : Math  Operator=square  SaturateOnIntegerOverflow=on
  Saturation : Saturate  UpperLimit=20  LowerLimit=0
  Saturation1 : Saturate  UpperLimit=500  LowerLimit=0
  Simulink-PS Converter : nesl_utility/Simulink-PS Converter  PhysicalDomain=network_engine_domain  SubClassName=ps_input  LeftPortType=input  RightPortType=output  PseudoPeriodic=off  Frequencies=[]  NoiseDistribution=none  NoiseParameters=[]  Unit=W  AffineConversion=on  FilteringAndDerivatives=provide  SimscapeFilterOrder=1  InputFilterTimeConstant=0.001  UdotUserProvided=0
  output : PMIOPort  Side=Left
  wires:
  In1/1 -> Saturation/1
  Saturation/1 -> Gain1/1
  Saturation1/1 -> Display1/1, Math Function/1
  Gain1/1 -> Saturation1/1
  Math Function/1 -> Gain2/1
  Gain2/1 -> Display/1, Simulink-PS Converter/1
  connections:
  output/RConn1 -- Simulink-PS Converter/RConn1

== matlab function SpeedGoatLoop_v2/MATLAB Function ==
  data: T input; dTdt output; valveCmd input; t input; Ts input; reset input; maxSlope output; ssThresh output; ssFlag output; ssTime output
function [dTdt, maxSlope, ssThresh, ssFlag, ssTime] = steadyStateMonitor(T, valveCmd, t, Ts, reset)
% valveCmd: 0 = closed, 1 = open
% reset: optional external reset

persistent Tprev maxSlopeLatch threshLatch ssTimer locked initialized firstRun

if isempty(initialized) || reset
    Tprev = T;
    maxSlopeLatch = 0;
    threshLatch = 0;
    ssTimer = 0;
    locked = false;
    initialized = true;
    
    firstRun = true;
end

% Discrete derivative
if firstRun
dTdt = 0;
firstRun = false;
else
    dTdt = (T- Tprev)/Ts;
end

Tprev = T;
%Ignore unrealistic startup spikes
if abs(dTdt) > 2
    dTdt = 0;
end

% Record max heating rate
%Ignore first 5 seconds to avoid initialization transient

if ~locked
    if t > 5 && t < 300
       if abs(dTdt) > maxSlopeLatch
           maxSlopeLatch = abs(dTdt);
       end
    elseif t >= 300
        if maxSlopeLatch > 0
        threshLatch = 0.01 * maxSlopeLatch;
        end
            locked = true;
    end
end

%Outputs
maxSlope = maxSlopeLatch;
ssThresh  = threshLatch;


% Duration under steady-state condition
if locked && abs(dTdt) <= ssThresh
    ssFlag = true;
    ssTimer = ssTimer + Ts;
else
    ssTimer = 0;   % change to "ssTimer = ssTimer + Ts;" if you want total time instead of consecutive time
    ssFlag = false;
end

ssTime = ssTimer;
end
